simulink library "ardupilot_custom_controller_lib"  (R2018b)
settings: Solver=VariableStepAuto  StartTime=0.0  StopTime=10.0  RelTol=1e-3
values from neighbouring files (symbols this model uses):
  log_config = repmat(log,1,num_batches_max)    [ardupilotInitLogMuxer.m]
settings Model: Creator=yannic  LastModifiedBy=yannic

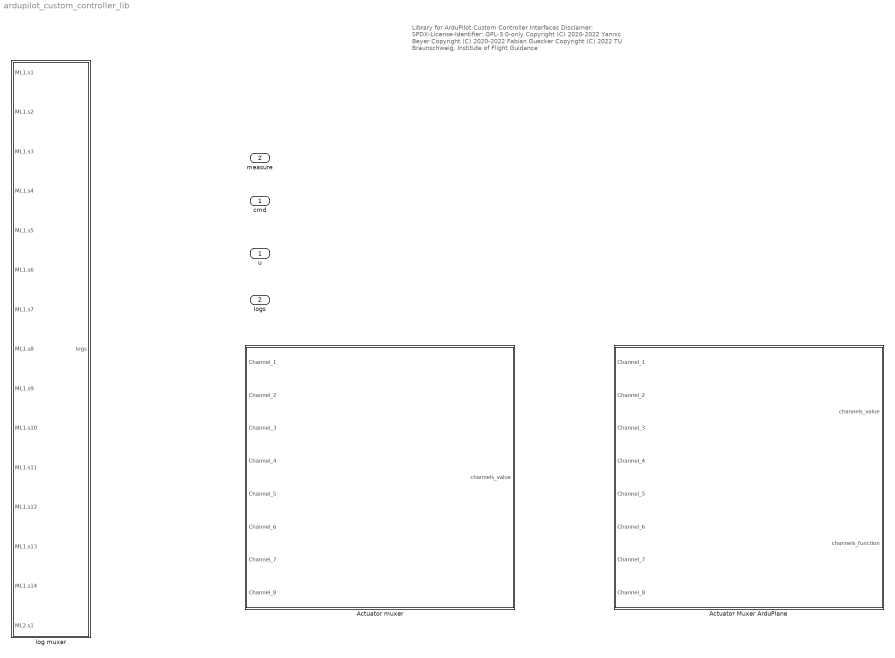
== system ardupilot_custom_controller_lib ==
  note: Library for ArduPilot Custom Controller Interfaces
      |
      | Disclamer:
      | SPDX-License-Identifier: GPL-3.0-only
      |
      | Copyright (C) 2020-2022 Yannic Beyer
      | Copyright (C) 2020-2022 Fabian Guecker
      | Copyright (C) 2022 TU Braunschweig, Institute of Flight Guidance
  cmd : Inport  OutDataTypeStr=Bus: cmdBus
  measure : Inport  Port=2  OutDataTypeStr=Bus: measureBus
  Actuator Muxer ArduPlane : Subsystem  mask{CHFCN1=k_aileron, CHFCN2=k_elevator, CHFCN3=k_throttle, CHFCN4=k_rudder, CHFCN5=k_none, CHFCN6=k_none, CHFCN7=k_none, CHFCN8=k_none}
      mask prompts: CHFCN1 "Function of channel 1"; CHFCN2 "Function of channel 2"; CHFCN3 "Function of channel 3"; CHFCN4 "Function of channel 4"; CHFCN5 "Function of channel 5"; CHFCN6 "Function of channel 6"; CHFCN7 "Function of channel 7"; CHFCN8 "Function of channel 8"
      mask TypeOptions CHFCN1: k_none | k_manual | k_flap | k_flap_auto | k_aileron | k_unused1 | k_mount_pan | k_mount_tilt | k_mount_roll | k_mount_open | k_cam_trigger | k_egg_drop | k_mount2_pan | k_mount2_tilt | k_mount2_roll | k_mount2_open | k_dspoilerLeft1 | k_dspoilerRight1 | k_aileron_with_input | k_elevator | k_elevator_with_input | k_rudder | k_sprayer_pump | k_sprayer_spinner | k_flaperon_left | k_flaperon_right | k_steering | k_parachute_release | k_gripper | k_landing_gear_control | k_engine_run_enable | k_heli_rsc | k_heli_tail_rsc | k_motor1 | k_motor2 | k_motor3 | k_motor4 | k_motor5 | k_motor6 | k_motor7 | k_motor8 | k_motor_tilt | k_generator_control | do-not-use-1 | do-not-use-2 | do-not-use-3 | do-not-use-4 | do-not-use-5 | do-not-use-6 | do-not-use-7 | do-not-use-8 | k_rcin1 | k_rcin2 | k_rcin3 | k_rcin4 | k_rcin5 | k_rcin6 | k_rcin7 | k_rcin8 | k_rcin9 | k_rcin10 | k_rcin11 | k_rcin12 | k_rcin13 | k_rcin14 | k_rcin15 | k_rcin16 | k_ignition | k_choke | k_starter | k_throttle | k_tracker_yaw | k_tracker_pitch | k_throttleLeft | k_throttleRight | k_tiltMotorLeft | k_tiltMotorRight | k_elevon_left | k_elevon_right | k_vtail_left | k_vtail_right | k_boost_throttle | k_motor9 | k_motor10 | k_motor11 | k_motor12 | k_dspoilerLeft2 | k_dspoilerRight2 | k_winch | k_mainsail_sheet | k_cam_iso | k_cam_aperture | k_cam_focus | k_cam_shutter_speed | k_scripting1 | k_scripting2 | k_scripting3 | k_scripting4 | k_scripting5 | k_scripting6 | k_scripting7 | k_scripting8 | k_scripting9 | k_scripting10 | k_scripting11 | k_scripting12 | k_scripting13 | k_scripting14 | k_scripting15 | k_scripting16 | k_airbrake | Do-not-use-9 | Do-not-use-10 | Do-not-use-11 | Do-not-use-12 | Do-not-use-13 | Do-not-use-14 | Do-not-use-15 | Do-not-use-16 | Do-not-use-17 | k_LED_neopixel1 | k_LED_neopixel2 | k_LED_neopixel3 | k_LED_neopixel4 | k_roll_out | k_pitch_out | k_thrust_out | k_yaw_out | k_wingsail_elevator | k_ProfiLED_1 | k_ProfiLED_2 | k_ProfiLED_3 | k_ProfiLED_Clock | k_winch_clutch
      mask TypeOptions CHFCN2: k_none | k_manual | k_flap | k_flap_auto | k_aileron | k_unused1 | k_mount_pan | k_mount_tilt | k_mount_roll | k_mount_open | k_cam_trigger | k_egg_drop | k_mount2_pan | k_mount2_tilt | k_mount2_roll | k_mount2_open | k_dspoilerLeft1 | k_dspoilerRight1 | k_aileron_with_input | k_elevator | k_elevator_with_input | k_rudder | k_sprayer_pump | k_sprayer_spinner | k_flaperon_left | k_flaperon_right | k_steering | k_parachute_release | k_gripper | k_landing_gear_control | k_engine_run_enable | k_heli_rsc | k_heli_tail_rsc | k_motor1 | k_motor2 | k_motor3 | k_motor4 | k_motor5 | k_motor6 | k_motor7 | k_motor8 | k_motor_tilt | k_generator_control | do-not-use-1 | do-not-use-2 | do-not-use-3 | do-not-use-4 | do-not-use-5 | do-not-use-6 | do-not-use-7 | do-not-use-8 | k_rcin1 | k_rcin2 | k_rcin3 | k_rcin4 | k_rcin5 | k_rcin6 | k_rcin7 | k_rcin8 | k_rcin9 | k_rcin10 | k_rcin11 | k_rcin12 | k_rcin13 | k_rcin14 | k_rcin15 | k_rcin16 | k_ignition | k_choke | k_starter | k_throttle | k_tracker_yaw | k_tracker_pitch | k_throttleLeft | k_throttleRight | k_tiltMotorLeft | k_tiltMotorRight | k_elevon_left | k_elevon_right | k_vtail_left | k_vtail_right | k_boost_throttle | k_motor9 | k_motor10 | k_motor11 | k_motor12 | k_dspoilerLeft2 | k_dspoilerRight2 | k_winch | k_mainsail_sheet | k_cam_iso | k_cam_aperture | k_cam_focus | k_cam_shutter_speed | k_scripting1 | k_scripting2 | k_scripting3 | k_scripting4 | k_scripting5 | k_scripting6 | k_scripting7 | k_scripting8 | k_scripting9 | k_scripting10 | k_scripting11 | k_scripting12 | k_scripting13 | k_scripting14 | k_scripting15 | k_scripting16 | k_airbrake | Do-not-use-9 | Do-not-use-10 | Do-not-use-11 | Do-not-use-12 | Do-not-use-13 | Do-not-use-14 | Do-not-use-15 | Do-not-use-16 | Do-not-use-17 | k_LED_neopixel1 | k_LED_neopixel2 | k_LED_neopixel3 | k_LED_neopixel4 | k_roll_out | k_pitch_out | k_thrust_out | k_yaw_out | k_wingsail_elevator | k_ProfiLED_1 | k_ProfiLED_2 | k_ProfiLED_3 | k_ProfiLED_Clock | k_winch_clutch
      mask TypeOptions CHFCN3: k_none | k_manual | k_flap | k_flap_auto | k_aileron | k_unused1 | k_mount_pan | k_mount_tilt | k_mount_roll | k_mount_open | k_cam_trigger | k_egg_drop | k_mount2_pan | k_mount2_tilt | k_mount2_roll | k_mount2_open | k_dspoilerLeft1 | k_dspoilerRight1 | k_aileron_with_input | k_elevator | k_elevator_with_input | k_rudder | k_sprayer_pump | k_sprayer_spinner | k_flaperon_left | k_flaperon_right | k_steering | k_parachute_release | k_gripper | k_landing_gear_control | k_engine_run_enable | k_heli_rsc | k_heli_tail_rsc | k_motor1 | k_motor2 | k_motor3 | k_motor4 | k_motor5 | k_motor6 | k_motor7 | k_motor8 | k_motor_tilt | k_generator_control | do-not-use-1 | do-not-use-2 | do-not-use-3 | do-not-use-4 | do-not-use-5 | do-not-use-6 | do-not-use-7 | do-not-use-8 | k_rcin1 | k_rcin2 | k_rcin3 | k_rcin4 | k_rcin5 | k_rcin6 | k_rcin7 | k_rcin8 | k_rcin9 | k_rcin10 | k_rcin11 | k_rcin12 | k_rcin13 | k_rcin14 | k_rcin15 | k_rcin16 | k_ignition | k_choke | k_starter | k_throttle | k_tracker_yaw | k_tracker_pitch | k_throttleLeft | k_throttleRight | k_tiltMotorLeft | k_tiltMotorRight | k_elevon_left | k_elevon_right | k_vtail_left | k_vtail_right | k_boost_throttle | k_motor9 | k_motor10 | k_motor11 | k_motor12 | k_dspoilerLeft2 | k_dspoilerRight2 | k_winch | k_mainsail_sheet | k_cam_iso | k_cam_aperture | k_cam_focus | k_cam_shutter_speed | k_scripting1 | k_scripting2 | k_scripting3 | k_scripting4 | k_scripting5 | k_scripting6 | k_scripting7 | k_scripting8 | k_scripting9 | k_scripting10 | k_scripting11 | k_scripting12 | k_scripting13 | k_scripting14 | k_scripting15 | k_scripting16 | k_airbrake | Do-not-use-9 | Do-not-use-10 | Do-not-use-11 | Do-not-use-12 | Do-not-use-13 | Do-not-use-14 | Do-not-use-15 | Do-not-use-16 | Do-not-use-17 | k_LED_neopixel1 | k_LED_neopixel2 | k_LED_neopixel3 | k_LED_neopixel4 | k_roll_out | k_pitch_out | k_thrust_out | k_yaw_out | k_wingsail_elevator | k_ProfiLED_1 | k_ProfiLED_2 | k_ProfiLED_3 | k_ProfiLED_Clock | k_winch_clutch
      mask TypeOptions CHFCN4: k_none | k_manual | k_flap | k_flap_auto | k_aileron | k_unused1 | k_mount_pan | k_mount_tilt | k_mount_roll | k_mount_open | k_cam_trigger | k_egg_drop | k_mount2_pan | k_mount2_tilt | k_mount2_roll | k_mount2_open | k_dspoilerLeft1 | k_dspoilerRight1 | k_aileron_with_input | k_elevator | k_elevator_with_input | k_rudder | k_sprayer_pump | k_sprayer_spinner | k_flaperon_left | k_flaperon_right | k_steering | k_parachute_release | k_gripper | k_landing_gear_control | k_engine_run_enable | k_heli_rsc | k_heli_tail_rsc | k_motor1 | k_motor2 | k_motor3 | k_motor4 | k_motor5 | k_motor6 | k_motor7 | k_motor8 | k_motor_tilt | k_generator_control | do-not-use-1 | do-not-use-2 | do-not-use-3 | do-not-use-4 | do-not-use-5 | do-not-use-6 | do-not-use-7 | do-not-use-8 | k_rcin1 | k_rcin2 | k_rcin3 | k_rcin4 | k_rcin5 | k_rcin6 | k_rcin7 | k_rcin8 | k_rcin9 | k_rcin10 | k_rcin11 | k_rcin12 | k_rcin13 | k_rcin14 | k_rcin15 | k_rcin16 | k_ignition | k_choke | k_starter | k_throttle | k_tracker_yaw | k_tracker_pitch | k_throttleLeft | k_throttleRight | k_tiltMotorLeft | k_tiltMotorRight | k_elevon_left | k_elevon_right | k_vtail_left | k_vtail_right | k_boost_throttle | k_motor9 | k_motor10 | k_motor11 | k_motor12 | k_dspoilerLeft2 | k_dspoilerRight2 | k_winch | k_mainsail_sheet | k_cam_iso | k_cam_aperture | k_cam_focus | k_cam_shutter_speed | k_scripting1 | k_scripting2 | k_scripting3 | k_scripting4 | k_scripting5 | k_scripting6 | k_scripting7 | k_scripting8 | k_scripting9 | k_scripting10 | k_scripting11 | k_scripting12 | k_scripting13 | k_scripting14 | k_scripting15 | k_scripting16 | k_airbrake | Do-not-use-9 | Do-not-use-10 | Do-not-use-11 | Do-not-use-12 | Do-not-use-13 | Do-not-use-14 | Do-not-use-15 | Do-not-use-16 | Do-not-use-17 | k_LED_neopixel1 | k_LED_neopixel2 | k_LED_neopixel3 | k_LED_neopixel4 | k_roll_out | k_pitch_out | k_thrust_out | k_yaw_out | k_wingsail_elevator | k_ProfiLED_1 | k_ProfiLED_2 | k_ProfiLED_3 | k_ProfiLED_Clock | k_winch_clutch
      mask TypeOptions CHFCN5: k_none | k_manual | k_flap | k_flap_auto | k_aileron | k_unused1 | k_mount_pan | k_mount_tilt | k_mount_roll | k_mount_open | k_cam_trigger | k_egg_drop | k_mount2_pan | k_mount2_tilt | k_mount2_roll | k_mount2_open | k_dspoilerLeft1 | k_dspoilerRight1 | k_aileron_with_input | k_elevator | k_elevator_with_input | k_rudder | k_sprayer_pump | k_sprayer_spinner | k_flaperon_left | k_flaperon_right | k_steering | k_parachute_release | k_gripper | k_landing_gear_control | k_engine_run_enable | k_heli_rsc | k_heli_tail_rsc | k_motor1 | k_motor2 | k_motor3 | k_motor4 | k_motor5 | k_motor6 | k_motor7 | k_motor8 | k_motor_tilt | k_generator_control | do-not-use-1 | do-not-use-2 | do-not-use-3 | do-not-use-4 | do-not-use-5 | do-not-use-6 | do-not-use-7 | do-not-use-8 | k_rcin1 | k_rcin2 | k_rcin3 | k_rcin4 | k_rcin5 | k_rcin6 | k_rcin7 | k_rcin8 | k_rcin9 | k_rcin10 | k_rcin11 | k_rcin12 | k_rcin13 | k_rcin14 | k_rcin15 | k_rcin16 | k_ignition | k_choke | k_starter | k_throttle | k_tracker_yaw | k_tracker_pitch | k_throttleLeft | k_throttleRight | k_tiltMotorLeft | k_tiltMotorRight | k_elevon_left | k_elevon_right | k_vtail_left | k_vtail_right | k_boost_throttle | k_motor9 | k_motor10 | k_motor11 | k_motor12 | k_dspoilerLeft2 | k_dspoilerRight2 | k_winch | k_mainsail_sheet | k_cam_iso | k_cam_aperture | k_cam_focus | k_cam_shutter_speed | k_scripting1 | k_scripting2 | k_scripting3 | k_scripting4 | k_scripting5 | k_scripting6 | k_scripting7 | k_scripting8 | k_scripting9 | k_scripting10 | k_scripting11 | k_scripting12 | k_scripting13 | k_scripting14 | k_scripting15 | k_scripting16 | k_airbrake | Do-not-use-9 | Do-not-use-10 | Do-not-use-11 | Do-not-use-12 | Do-not-use-13 | Do-not-use-14 | Do-not-use-15 | Do-not-use-16 | Do-not-use-17 | k_LED_neopixel1 | k_LED_neopixel2 | k_LED_neopixel3 | k_LED_neopixel4 | k_roll_out | k_pitch_out | k_thrust_out | k_yaw_out | k_wingsail_elevator | k_ProfiLED_1 | k_ProfiLED_2 | k_ProfiLED_3 | k_ProfiLED_Clock | k_winch_clutch
      mask TypeOptions CHFCN6: k_none | k_manual | k_flap | k_flap_auto | k_aileron | k_unused1 | k_mount_pan | k_mount_tilt | k_mount_roll | k_mount_open | k_cam_trigger | k_egg_drop | k_mount2_pan | k_mount2_tilt | k_mount2_roll | k_mount2_open | k_dspoilerLeft1 | k_dspoilerRight1 | k_aileron_with_input | k_elevator | k_elevator_with_input | k_rudder | k_sprayer_pump | k_sprayer_spinner | k_flaperon_left | k_flaperon_right | k_steering | k_parachute_release | k_gripper | k_landing_gear_control | k_engine_run_enable | k_heli_rsc | k_heli_tail_rsc | k_motor1 | k_motor2 | k_motor3 | k_motor4 | k_motor5 | k_motor6 | k_motor7 | k_motor8 | k_motor_tilt | k_generator_control | do-not-use-1 | do-not-use-2 | do-not-use-3 | do-not-use-4 | do-not-use-5 | do-not-use-6 | do-not-use-7 | do-not-use-8 | k_rcin1 | k_rcin2 | k_rcin3 | k_rcin4 | k_rcin5 | k_rcin6 | k_rcin7 | k_rcin8 | k_rcin9 | k_rcin10 | k_rcin11 | k_rcin12 | k_rcin13 | k_rcin14 | k_rcin15 | k_rcin16 | k_ignition | k_choke | k_starter | k_throttle | k_tracker_yaw | k_tracker_pitch | k_throttleLeft | k_throttleRight | k_tiltMotorLeft | k_tiltMotorRight | k_elevon_left | k_elevon_right | k_vtail_left | k_vtail_right | k_boost_throttle | k_motor9 | k_motor10 | k_motor11 | k_motor12 | k_dspoilerLeft2 | k_dspoilerRight2 | k_winch | k_mainsail_sheet | k_cam_iso | k_cam_aperture | k_cam_focus | k_cam_shutter_speed | k_scripting1 | k_scripting2 | k_scripting3 | k_scripting4 | k_scripting5 | k_scripting6 | k_scripting7 | k_scripting8 | k_scripting9 | k_scripting10 | k_scripting11 | k_scripting12 | k_scripting13 | k_scripting14 | k_scripting15 | k_scripting16 | k_airbrake | Do-not-use-9 | Do-not-use-10 | Do-not-use-11 | Do-not-use-12 | Do-not-use-13 | Do-not-use-14 | Do-not-use-15 | Do-not-use-16 | Do-not-use-17 | k_LED_neopixel1 | k_LED_neopixel2 | k_LED_neopixel3 | k_LED_neopixel4 | k_roll_out | k_pitch_out | k_thrust_out | k_yaw_out | k_wingsail_elevator | k_ProfiLED_1 | k_ProfiLED_2 | k_ProfiLED_3 | k_ProfiLED_Clock | k_winch_clutch
      mask TypeOptions CHFCN7: k_none | k_manual | k_flap | k_flap_auto | k_aileron | k_unused1 | k_mount_pan | k_mount_tilt | k_mount_roll | k_mount_open | k_cam_trigger | k_egg_drop | k_mount2_pan | k_mount2_tilt | k_mount2_roll | k_mount2_open | k_dspoilerLeft1 | k_dspoilerRight1 | k_aileron_with_input | k_elevator | k_elevator_with_input | k_rudder | k_sprayer_pump | k_sprayer_spinner | k_flaperon_left | k_flaperon_right | k_steering | k_parachute_release | k_gripper | k_landing_gear_control | k_engine_run_enable | k_heli_rsc | k_heli_tail_rsc | k_motor1 | k_motor2 | k_motor3 | k_motor4 | k_motor5 | k_motor6 | k_motor7 | k_motor8 | k_motor_tilt | k_generator_control | do-not-use-1 | do-not-use-2 | do-not-use-3 | do-not-use-4 | do-not-use-5 | do-not-use-6 | do-not-use-7 | do-not-use-8 | k_rcin1 | k_rcin2 | k_rcin3 | k_rcin4 | k_rcin5 | k_rcin6 | k_rcin7 | k_rcin8 | k_rcin9 | k_rcin10 | k_rcin11 | k_rcin12 | k_rcin13 | k_rcin14 | k_rcin15 | k_rcin16 | k_ignition | k_choke | k_starter | k_throttle | k_tracker_yaw | k_tracker_pitch | k_throttleLeft | k_throttleRight | k_tiltMotorLeft | k_tiltMotorRight | k_elevon_left | k_elevon_right | k_vtail_left | k_vtail_right | k_boost_throttle | k_motor9 | k_motor10 | k_motor11 | k_motor12 | k_dspoilerLeft2 | k_dspoilerRight2 | k_winch | k_mainsail_sheet | k_cam_iso | k_cam_aperture | k_cam_focus | k_cam_shutter_speed | k_scripting1 | k_scripting2 | k_scripting3 | k_scripting4 | k_scripting5 | k_scripting6 | k_scripting7 | k_scripting8 | k_scripting9 | k_scripting10 | k_scripting11 | k_scripting12 | k_scripting13 | k_scripting14 | k_scripting15 | k_scripting16 | k_airbrake | Do-not-use-9 | Do-not-use-10 | Do-not-use-11 | Do-not-use-12 | Do-not-use-13 | Do-not-use-14 | Do-not-use-15 | Do-not-use-16 | Do-not-use-17 | k_LED_neopixel1 | k_LED_neopixel2 | k_LED_neopixel3 | k_LED_neopixel4 | k_roll_out | k_pitch_out | k_thrust_out | k_yaw_out | k_wingsail_elevator | k_ProfiLED_1 | k_ProfiLED_2 | k_ProfiLED_3 | k_ProfiLED_Clock | k_winch_clutch
      mask TypeOptions CHFCN8: k_none | k_manual | k_flap | k_flap_auto | k_aileron | k_unused1 | k_mount_pan | k_mount_tilt | k_mount_roll | k_mount_open | k_cam_trigger | k_egg_drop | k_mount2_pan | k_mount2_tilt | k_mount2_roll | k_mount2_open | k_dspoilerLeft1 | k_dspoilerRight1 | k_aileron_with_input | k_elevator | k_elevator_with_input | k_rudder | k_sprayer_pump | k_sprayer_spinner | k_flaperon_left | k_flaperon_right | k_steering | k_parachute_release | k_gripper | k_landing_gear_control | k_engine_run_enable | k_heli_rsc | k_heli_tail_rsc | k_motor1 | k_motor2 | k_motor3 | k_motor4 | k_motor5 | k_motor6 | k_motor7 | k_motor8 | k_motor_tilt | k_generator_control | do-not-use-1 | do-not-use-2 | do-not-use-3 | do-not-use-4 | do-not-use-5 | do-not-use-6 | do-not-use-7 | do-not-use-8 | k_rcin1 | k_rcin2 | k_rcin3 | k_rcin4 | k_rcin5 | k_rcin6 | k_rcin7 | k_rcin8 | k_rcin9 | k_rcin10 | k_rcin11 | k_rcin12 | k_rcin13 | k_rcin14 | k_rcin15 | k_rcin16 | k_ignition | k_choke | k_starter | k_throttle | k_tracker_yaw | k_tracker_pitch | k_throttleLeft | k_throttleRight | k_tiltMotorLeft | k_tiltMotorRight | k_elevon_left | k_elevon_right | k_vtail_left | k_vtail_right | k_boost_throttle | k_motor9 | k_motor10 | k_motor11 | k_motor12 | k_dspoilerLeft2 | k_dspoilerRight2 | k_winch | k_mainsail_sheet | k_cam_iso | k_cam_aperture | k_cam_focus | k_cam_shutter_speed | k_scripting1 | k_scripting2 | k_scripting3 | k_scripting4 | k_scripting5 | k_scripting6 | k_scripting7 | k_scripting8 | k_scripting9 | k_scripting10 | k_scripting11 | k_scripting12 | k_scripting13 | k_scripting14 | k_scripting15 | k_scripting16 | k_airbrake | Do-not-use-9 | Do-not-use-10 | Do-not-use-11 | Do-not-use-12 | Do-not-use-13 | Do-not-use-14 | Do-not-use-15 | Do-not-use-16 | Do-not-use-17 | k_LED_neopixel1 | k_LED_neopixel2 | k_LED_neopixel3 | k_LED_neopixel4 | k_roll_out | k_pitch_out | k_thrust_out | k_yaw_out | k_wingsail_elevator | k_ProfiLED_1 | k_ProfiLED_2 | k_ProfiLED_3 | k_ProfiLED_Clock | k_winch_clutch
      mask DialogControl DescGroupVar Prompt: Actuator output muxer
      mask DialogControl DescTextVar Prompt: Connect the actuator signal (0...1) to the corresponding port.
      mask Display:
      | port_label('input',1,get_param(gcb,'CHFCN1'));
      | port_label('input',2,get_param(gcb,'CHFCN2'));
      | port_label('input',3,get_param(gcb,'CHFCN3'));
      | port_label('input',4,get_param(gcb,'CHFCN4'));
      | port_label('input',5,get_param(gcb,'CHFCN5'));
      | port_label('input',6,get_param(gcb,'CHFCN6'));
      | port_label('input',7,get_param(gcb,'CHFCN7'));
      | port_label('input',8,get_param(gcb,'CHFCN8'));
      | 
      | port_label('output',1,'channels');
      | port_label('output',2,'function_channels');
  Actuator muxer : Subsystem
      mask DialogControl DescGroupVar Prompt: Actuator muxer
  log muxer : Subsystem  mask{batch_name_1='ML1', num_signals_1=14, batch_name_2='ML2', num_signals_2=1, batch_name_3='ML3', num_signals_3=0, batch_name_4='ML4', num_signals_4=0, batch_name_5='ML5', num_signals_5=0}
      mask prompts: batch_name_1 "Name (max. 4 characters)"; num_signals_1 "Number of signals (0 ... 14)"; batch_name_2 "Name (max. 4 characters)"; num_signals_2 "Number of signals (0 ... 14)"; batch_name_3 "Name (max. 4 characters)"; num_signals_3 "Number of signals (0 ... 14)"; batch_name_4 "Name (max. 4 characters)"; num_signals_4 "Number of signals (0 ... 14)"; batch_name_5 "Name (max. 4 characters)"; num_signals_5 "Number of signals (0 ... 14)"
      mask init:
      | batch_name_in = { batch_name_1, batch_name_2, batch_name_3, batch_name_4, batch_name_5 };
      | num_signals_in = [ num_signals_1, num_signals_2, num_signals_3, num_signals_4, num_signals_5 ];
      | ardupilotInitLogMuxer(gcb,batch_name_in,num_signals_in);
      mask DialogControl DescGroupVar Prompt: ArduPilot log muxer
      mask DialogControl DescTextVar Prompt: Assign signals to be logged in ArduPilot. If you haven't already, familiarize yourself with the format of ArduPilot logs:
      mask DialogControl Control3 Prompt: ArduPilot: Adding a new Log Message
      mask DialogControl Control3 Callback: web('https://ardupilot.org/dev/docs/code-overview-adding-a-new-log-message.html','-browser')
      mask DialogControl Control2 Prompt: In the block mask you can specify up to five "batch names" with each up to 14 signals. The signal names will automatically be adjusted if you provide a signal name for each connected signal (only 3 characters can be taken). The number of inports of the block will change automatically if you touch the number of signals in the mask.
      mask DialogControl group_1 Prompt: 1st batch:
      mask DialogControl group_2 Prompt: 2nd batch:
      mask DialogControl group_3 Prompt: 3rd batch:
      mask DialogControl group_4 Prompt: 4th batch:
      mask DialogControl group_5 Prompt: 5th batch:
  u : Outport
  logs : Outport  Port=2

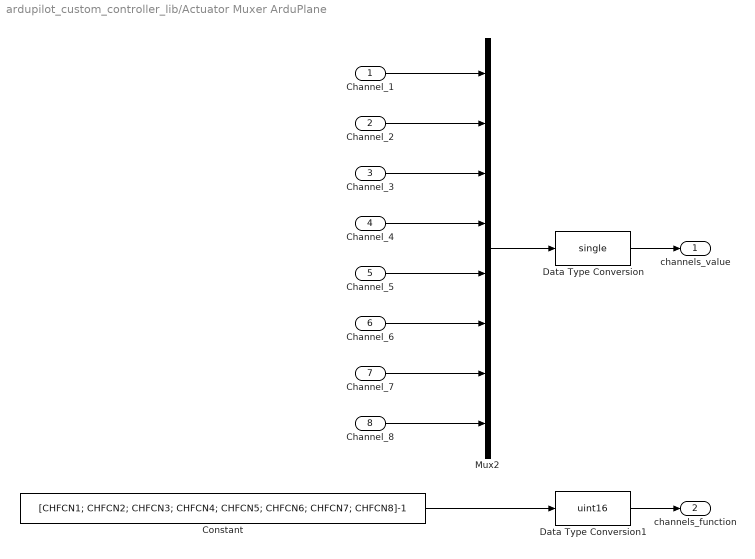
== system ardupilot_custom_controller_lib/Actuator Muxer ArduPlane ==
  Channel_1 : Inport
  Channel_2 : Inport  Port=2
  Channel_3 : Inport  Port=3
  Channel_4 : Inport  Port=4
  Channel_5 : Inport  Port=5
  Channel_6 : Inport  Port=6
  Channel_7 : Inport  Port=7
  Channel_8 : Inport  Port=8
  Constant : Constant  Value=[CHFCN1; CHFCN2; CHFCN3; CHFCN4; CHFCN5; CHFCN6; CHFCN7; CHFCN8]-1
  Data Type Conversion : DataTypeConversion  OutDataTypeStr=single
  Data Type Conversion1 : DataTypeConversion  OutDataTypeStr=uint16
  Mux2 : Mux  Inputs=8
  channels_value : Outport  OutDataTypeStr=single
  channels_function : Outport  Port=2  OutDataTypeStr=uint16
  wires:
  Channel_6/1 -> Mux2/6
  Channel_3/1 -> Mux2/3
  Channel_8/1 -> Mux2/8
  Channel_5/1 -> Mux2/5
  Channel_7/1 -> Mux2/7
  Mux2/1 -> Data Type Conversion/1
  Channel_1/1 -> Mux2/1
  Channel_4/1 -> Mux2/4
  Channel_2/1 -> Mux2/2
  Data Type Conversion/1 -> channels_value/1
  Data Type Conversion1/1 -> channels_function/1
  Constant/1 -> Data Type Conversion1/1

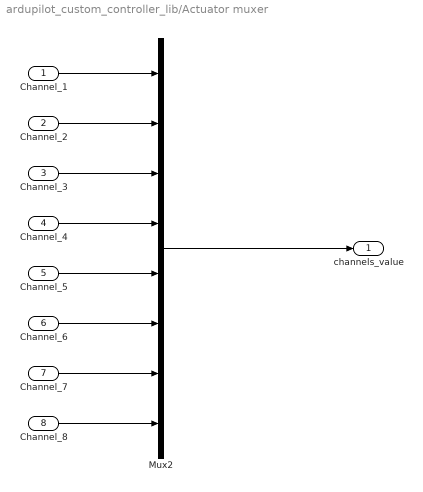
== system ardupilot_custom_controller_lib/Actuator muxer ==
  Channel_1 : Inport
  Channel_2 : Inport  Port=2
  Channel_3 : Inport  Port=3
  Channel_4 : Inport  Port=4
  Channel_5 : Inport  Port=5
  Channel_6 : Inport  Port=6
  Channel_7 : Inport  Port=7
  Channel_8 : Inport  Port=8
  Mux2 : Mux  Inputs=8
  channels_value : Outport
  wires:
  Channel_6/1 -> Mux2/6
  Channel_3/1 -> Mux2/3
  Channel_8/1 -> Mux2/8
  Channel_5/1 -> Mux2/5
  Channel_7/1 -> Mux2/7
  Channel_1/1 -> Mux2/1
  Channel_4/1 -> Mux2/4
  Channel_2/1 -> Mux2/2
  Mux2/1 -> channels_value/1

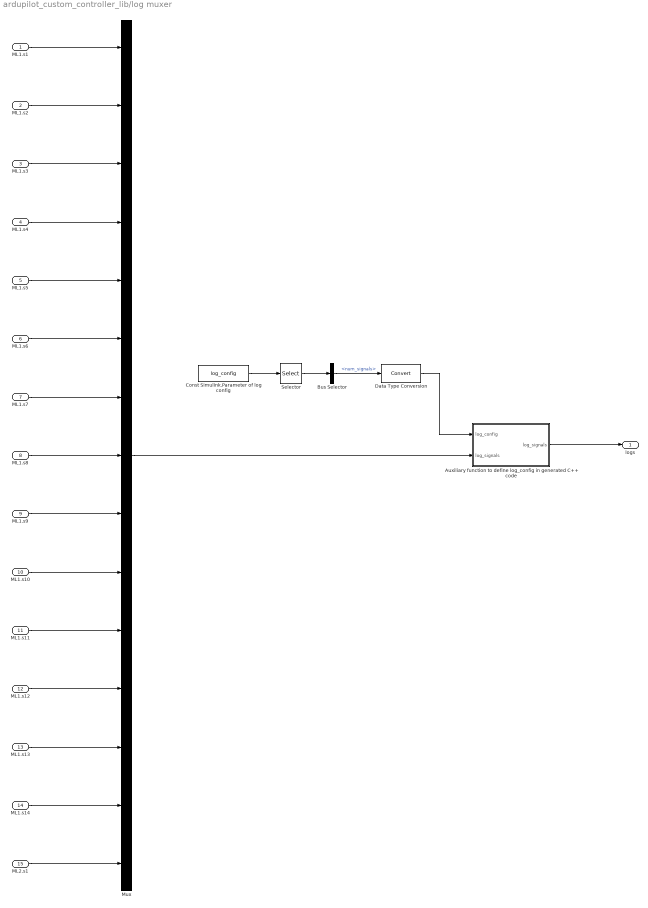
== system ardupilot_custom_controller_lib/log muxer ==
  ML1.s1 : Inport
  ML1.s2 : Inport  Port=2
  ML1.s3 : Inport  Port=3
  ML1.s4 : Inport  Port=4
  ML1.s5 : Inport  Port=5
  ML1.s6 : Inport  Port=6
  ML1.s7 : Inport  Port=7
  ML1.s8 : Inport  Port=8
  ML1.s9 : Inport  Port=9
  ML1.s10 : Inport  Port=10
  ML1.s11 : Inport  Port=11
  ML1.s12 : Inport  Port=12
  ML1.s13 : Inport  Port=13
  ML1.s14 : Inport  Port=14
  ML2.s1 : Inport  Port=15
  Auxiliary function to define log_config in generated C++ code : MATLAB Function  TreatAsAtomicUnit=on
  Bus Selector : BusSelector  OutputSignals=num_signals
  Const Simulink.Parameter of log config : Constant  Value=log_config  OutDataTypeStr=Bus: logConfigBus
  Data Type Conversion : DataTypeConversion
  Mux : Mux  Inputs=15
  Selector : Selector  InputPortWidth=length(batch_name_in)  IndexOptions=Index vector (dialog)  Indices=1  OutputSizes=1
  logs : Outport
  wires:
  Const Simulink.Parameter of log config/1 -> Selector/1
  Selector/1 -> Bus Selector/1
  Mux/1 -> Auxiliary function to define log_config in generated C++ code/2("log_signals ")
  Bus Selector/1 -> Data Type Conversion/1  "<num_signals>"
  Auxiliary function to define log_config in generated C++ code/1(log_signals) -> logs/1
  Data Type Conversion/1 -> Auxiliary function to define log_config in generated C++ code/1(log_config)
  ML1.s1/1 -> Mux/1
  ML1.s2/1 -> Mux/2
  ML1.s3/1 -> Mux/3
  ML1.s4/1 -> Mux/4
  ML1.s5/1 -> Mux/5
  ML1.s6/1 -> Mux/6
  ML1.s7/1 -> Mux/7
  ML1.s8/1 -> Mux/8
  ML1.s9/1 -> Mux/9
  ML1.s10/1 -> Mux/10
  ML1.s11/1 -> Mux/11
  ML1.s12/1 -> Mux/12
  ML1.s13/1 -> Mux/13
  ML1.s14/1 -> Mux/14
  ML2.s1/1 -> Mux/15

== matlab function ardupilot_custom_controller_lib/log muxer/Auxiliary function to define log_config in generated C++ code ==
  data: log_config input; log_signals input; log_signals output
function log_signals = fcn(log_config, log_signals)
end
